simulink model "FMT_QuadPlant"  (R2026b)
settings: Solver=FixedStepDiscrete  StopTime=2  FixedStep=0.0005
undefined symbols (not defined in the file): PlantState0, PlantStepS
settings Model: DataDictionary=Flight_Parameters.sldd  Creator=26718  LastModifiedBy=26718

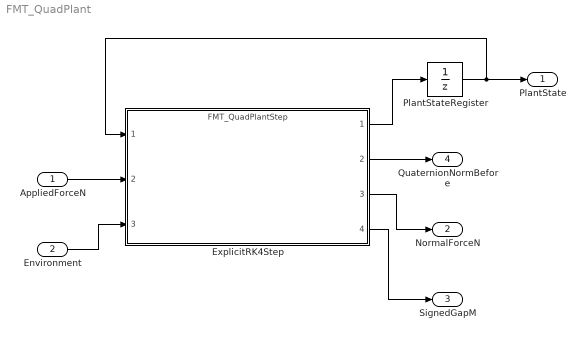
== system FMT_QuadPlant ==
  AppliedForceN : Inport  OutDataTypeStr=double  PortDimensions=4
  Environment : Inport  Port=2  OutDataTypeStr=double  PortDimensions=15
  ExplicitRK4Step : ModelReference  ModelNameDialog=FMT_QuadPlantStep  SimulationMode=Normal  ModelReferenceVersion=1.1
  PlantStateRegister : UnitDelay  InitialCondition=PlantState0  SampleTime=PlantStepS
  PlantState : Outport
  NormalForceN : Outport  Port=2
  SignedGapM : Outport  Port=3
  QuaternionNormBefore : Outport  Port=4
  wires:
  ExplicitRK4Step/4 -> SignedGapM/1
  ExplicitRK4Step/3 -> NormalForceN/1
  ExplicitRK4Step/2 -> QuaternionNormBefore/1
  ExplicitRK4Step/1 -> PlantStateRegister/1
  Environment/1 -> ExplicitRK4Step/3
  AppliedForceN/1 -> ExplicitRK4Step/2
  PlantStateRegister/1 -> ExplicitRK4Step/1, PlantState/1
